simulink model "surrogate_model_15"  (R2026a)
settings: Solver=VariableStepAuto
settings Model: Creator=shuki  LastModifiedBy=shuki

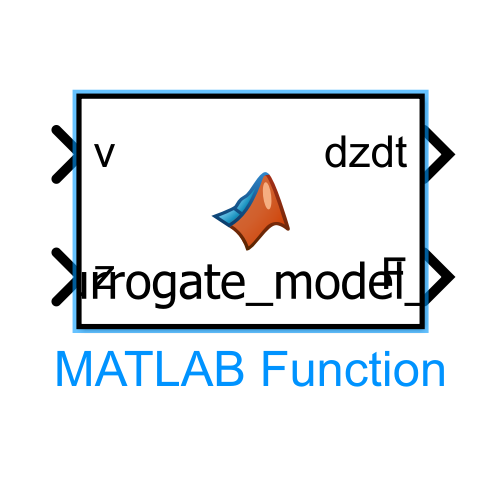
[thumbnail: Simulink's stored preview of the top-level diagram]
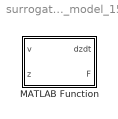
== system surrogate_model_15 ==
  MATLAB Function : MATLAB Function  TreatAsAtomicUnit=on

== matlab function surrogate_model_15/MATLAB Function ==
  data: dzdt output; F output; v input; z input
function [dzdt, F] = surrogate_model_15(v, z)

    S0 = 10^5;
    C1 = 0.00042237472;
    C2 = 2.807613;

    dzdt = v - abs(v)*(S0*z - ((S0*z) / (S0^2*abs(v)*abs(C1*v) + C2)));

    F = 10^5 * z + 316.2277 * dzdt + 0.4 * v;

end
